simulink model "Differentiator0"  (R2026a)
settings: Solver=ode4  StopTime=tf  FixedStep=0.01
values from neighbouring files (symbols this model uses):
  Differentiator = struct('G1', G1 ,     'G2', G2 ,     'Q1', Q1 ,     'Q2', Q2 ,     'w1', w1 ,     'w2', w2 ,     'p1', p1 ,     'p2', p2)    [init_model.m]    (also in init_var.m)
settings Model: SILPILSystemUnderTest=refmodels  Creator=Carlos Fabian  LastModifiedBy=Carlos Fabian
settings OptimizationCC: UseDivisionForNetSlopeComputation=on  GainParamInheritBuiltInType=on  UseFloatMulNetSlope=on  InlineInvariantSignals=on  EfficientFloat2IntCast=on
settings RTWCC: SystemTargetFile=ert.tlc  GenerateReport=on  LaunchReport=on  TargetLang=C++  Description=Embedded Coder
settings ERTTargetCC: RootIOFormat=Structure reference  TargetLangStandard=C++11 (ISO)  GenerateSampleERTMain=on  CodeInterfacePackaging=C++ class  SubcomponentCodeInterfacePackaging=C++ class  SupportContinuousTime=on
settings ExplorerConfigSet: InternalSimMechanicsExplorerSettings=|
  | <ExplorerConfiguration>
  | 
  |   <canonicalview>default</canonicalview>
  | 
  |   <TilePanel>
  |     <TileInfo>
  |       <Tiles Columns="1" Count="1" Height="513" Rows="1" Width="1199">
  |         <Row Weight="1"/>
  |         <Column Weight="1"/>
  |         <Tile Height="1" Width="1" X="0" Y="0"/>
  |       </Tiles>
  |     </TileInfo>
  |     <SceneInfo>
  |       <SceneViewer>
  |         <IsThisViewStd>
  |           <IsStandardView>off</IsStandardView>
  |           <StandardViewName>Front</StandardViewName>
  |         </IsThisViewStd>
  |         <BGColor>
  |           <R>1</R>
  |           <G>1</G>
  |           <B>1</B>
  |           <A>1</A>
  |         </BGColor>
  |         <Camera>
  |           <DoPerspective>off</DoPerspective>
  |           <Position>
  |             <X>16.563809413425133</X>
  |             <Y>-16.563809413425133</Y>
  |             <Z>17.346953838391503</Z>
  |           </Position>
  |           <Center>
  |             <X>0</X>
  |             <Y>0</Y>
  |             <Z>0.78314442496637693</Z>
  |           </Center>
  |           <Up>
  |             <X>-0.40824829046386285</X>
  |             <Y>0.40824829046386285</Y>
  |             <Z>0.81649658092772603</Z>
  |           </Up>
  |           <XLim>3.39184009237395</XLim>
  |           <YLim>3.39184009237395</YLim>
  |           <ViewLimDist>0.01</ViewLimDist>
  |         </Camera>
  |       </SceneViewer>
  |     </SceneInfo>
  |   </TilePanel>
  | 
  |   <MechEditorPanel>
  |     <GfxPanelCameraMap/>
  |     <Cameras/>
  |     <VideoCreator>
  |       <IncludeTiles>All</IncludeTiles>
  |       <IncludeTime>on</IncludeTime>
  |       <IncludeWorldFrame>off</IncludeWorldFrame>
  |       <PlaybackSpeedRatio>8</PlaybackSpeedRatio>
  |       <FrameRate>24</FrameRate>
  |       <FrameSize>auto</FrameSize>
  |       <VideoFormat>MotionJPEGAVI</VideoFormat>
  |     </VideoCreator>
  |   </MechEditorPanel>
  | 
  |   <PlaybackSettings>
  |     <PlaybackSpeedFactor>4</PlaybackSpeedFactor>
  |   </PlaybackSettings>
  | 
  | </ExplorerConfiguration>

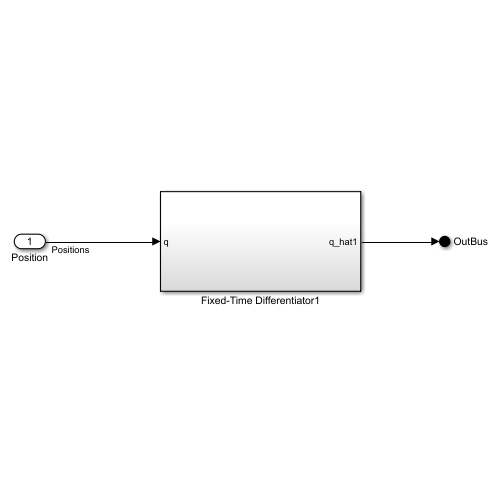
[thumbnail: Simulink's stored preview of the top-level diagram]
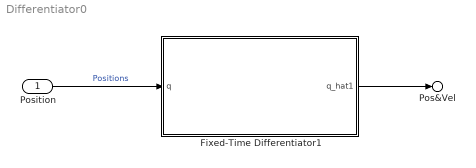
== system Differentiator0 ==
  Position : Inport  OutDataTypeStr=double  PortDimensions=8  SampleTime=0
  Fixed-Time Differentiator1 : Subsystem
      settings: PortSchema="{\"entries\":[{\"content\":{\"sides\":[{\"content\":{\"connectorIds\":[\"Out1\"]},\"type\":\"ConnectorPlacement.EquallySpacedRectSide\",\"uuid\":\"d79ec49c-5563-41e0-ac59-6e897bc19fda\"},{\"content\":{\"connectorIds\":[\"In1\"],\"side\":\"RIGHT\"},\"type\":\"ConnectorPlacement.EquallySpacedRectSide\",\"uuid\":\"1255043e-c90e-4bae-9fb4-4fa06f36f53e\"},{\"content\":{\"side\":\"TOP\"},\"type\":\"ConnectorPlacement.EquallySpacedRectSide\",\"uuid\":\"823ada36-3f22-4ee3-87a1-180276f622bc\"}]},\"type\":\"ConnectorPlacement.EquallySpacedConnector\",\"uuid\":\"7403b609-b333-4977-a854-ed7a71f74338\"}],\"packageUris\":[\"http://schema.mathworks.com/mf0/Connector/R2020b\"],\"version\":\"1.0\"}"
  Pos&Vel : Outport  PortName=OutBus
  wires:
  Position/1 -> Fixed-Time Differentiator1/1(q)  "Positions"
  Fixed-Time Differentiator1/1(q_hat1) -> Pos&Vel/1

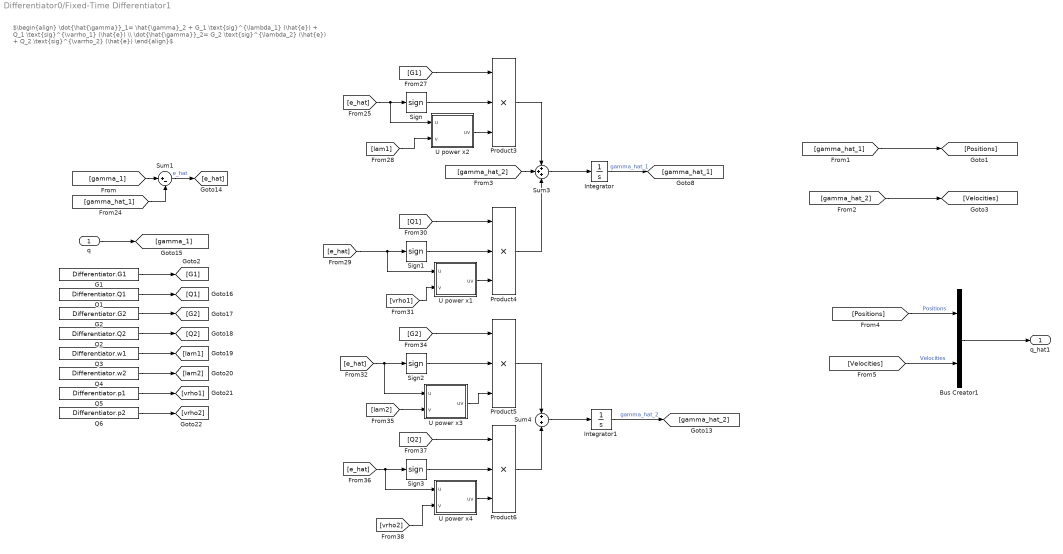
== system Differentiator0/Fixed-Time Differentiator1 ==
  note: $\begin{align} \dot{\hat{\gamma}}_1= \hat{\gamma}_2 + G_1 \text{sig}^{\lambda_1} (\hat{e}) + Q_1 \text{sig}^{\varrho_1} (\hat{e}) \\ \dot{\hat{\gamma}}_2= G_2 \text{sig}^{\lambda_2} (\hat{e}) + Q_2 \text{sig}^{\varrho_2} (\hat{e}) \end{align}$
  q : Inport
  Bus Creator1 : BusCreator  Inputs=2
  G1 : Constant  Value=Differentiator.G1
  G2 : Constant  Value=Differentiator.G2
  Integrator : Integrator  InitialCondition=[0; 0; 0.28; 0; 0; 0; 0; 0]  IgnoreLimit=on
  Integrator1 : Integrator  InitialCondition=[0; 0; 0; 0; 0; 0; 0; 0]  IgnoreLimit=on
  Product{3..6} (4 alike) : Product  Inputs=3
  Q1 : Constant  Value=Differentiator.Q1
  Q2 : Constant  Value=Differentiator.Q2
  Q3 : Constant  Value=Differentiator.w1
  Q4 : Constant  Value=Differentiator.w2
  Q5 : Constant  Value=Differentiator.p1
  Q6 : Constant  Value=Differentiator.p2
  Sign{,1..3} (4 alike) : Signum
  Sum1 : Sum  Inputs=|+-
  Sum3 : Sum  Inputs=+++
  Sum4 : Sum  Inputs=+|+
  U power x1 : MATLAB Function  TreatAsAtomicUnit=on
  U power x2 : MATLAB Function  TreatAsAtomicUnit=on
  U power x3 : MATLAB Function  TreatAsAtomicUnit=on
  U power x4 : MATLAB Function  TreatAsAtomicUnit=on
  q_hat1 : Outport
  wires:
  Integrator1/1 -> [gamma_hat_2]  "gamma_hat_2"
  [Velocities] -> Bus Creator1/2  "Velocities"
  [Positions] -> Bus Creator1/1  "Positions"
  Bus Creator1/1 -> q_hat1/1
  [gamma_hat_1] -> [Positions]
  U power x4/1(uv) -> Product6/3
  U power x3/1(uv) -> Product5/3
  U power x1/1(uv) -> Product4/3
  [lam1] -> U power x2/2(v)
  U power x2/1(uv) -> Product3/3
  [e_hat] -> Sign/1, U power x2/1(u)
  [e_hat] -> Sign3/1, U power x4/1(u)
  [e_hat] -> Sign2/1, U power x3/1(u)
  [e_hat] -> Sign1/1, U power x1/1(u)
  [Q1] -> Product4/1
  [vrho1] -> U power x1/2(v)
  Sign1/1 -> Product4/2
  Product4/1 -> Sum3/3
  [gamma_hat_2] -> Sum3/2
  Sum3/1 -> Integrator/1
  Sum4/1 -> Integrator1/1
  [gamma_hat_2] -> [Velocities]
  Integrator/1 -> [gamma_hat_1]  "gamma_hat_1"
  q/1 -> [gamma_1]
  Q3/1 -> [lam1]
  Sign/1 -> Product3/2
  Product3/1 -> Sum3/1
  [Q2] -> Product6/1
  [G2] -> Product5/1
  [lam2] -> U power x3/2(v)
  [gamma_1] -> Sum1/1
  Product5/1 -> Sum4/1
  Q4/1 -> [lam2]
  Sign2/1 -> Product5/2
  G2/1 -> [G2]
  [G1] -> Product3/1
  Q2/1 -> [Q2]
  [vrho2] -> U power x4/2(v)
  Q6/1 -> [vrho2]
  Q1/1 -> [Q1]
  Q5/1 -> [vrho1]
  [gamma_hat_1] -> Sum1/2
  Sign3/1 -> Product6/2
  Sum1/1 -> [e_hat]  "e_hat"
  G1/1 -> [G1]
  Product6/1 -> Sum4/2

== matlab function Differentiator0/Fixed-Time Differentiator1/U power x1 ==
  data: u input; uv output; v input
function uv = u_x(u, v)
i = 1;
uv = zeros(8,1);
for i=1:8
    absolute = abs(u(i));
    uv(i) = absolute ^ v(i);
    % if absolute < 0.00005
    %     uv(i) = 0;
    % else
    %     uv(i) = absolute ^ v(i);
    % end
end
end

== matlab function Differentiator0/Fixed-Time Differentiator1/U power x3 ==
  data: u input; uv output; v input
function uv = u_x(u, v)
i = 1;
uv = zeros(8,1);
for i=1:8
    absolute = abs(u(i));
    uv(i) = absolute ^ v(i);
    % if absolute < 0.00005
    %     uv(i) = 0;
    % else
    %     uv(i) = absolute ^ v(i);
    % end
end
end

== matlab function Differentiator0/Fixed-Time Differentiator1/U power x4 ==
  data: u input; uv output; v input
function uv = u_x(u, v)
i = 1;
uv = zeros(8,1);
for i=1:8
    absolute = abs(u(i));
    uv(i) = absolute ^ v(i);
    % if absolute < 0.00005
    %     uv(i) = 0;
    % else
    %     uv(i) = absolute ^ v(i);
    % end
end
end

== matlab function Differentiator0/Fixed-Time Differentiator1/U power x2 ==
  data: u input; uv output; v input
function uv = u_x(u, v)
i = 1;
uv = zeros(8,1);
for i=1:8
    absolute = abs(u(i));
    uv(i) = absolute ^ v(i);
    % if absolute < 0.00005
    %     uv(i) = 0;
    % else
    %     uv(i) = absolute ^ v(i);
    % end
end
end
